simulink model "snap_adc5g_spec"  (R2019a)
settings: Solver=VariableStepDiscrete  StartTime=0.0  StopTime=10.0  RelTol=1e-3
undefined symbols (not defined in the file): pfb_coeff_gen_calc
libraries: xbsIndex_r4 x13965, casper_library_misc x80, casper_library_delays x43, xps_library x5, xbsReplacements_r4 x2, casper_library_communications x1
(part 152 of 152)

== system snap_adc5g_spec/fft_wideband_real/fft_biplex_real_4x/biplex_core/fft_stage_11/butterfly_direct/twiddle/bus_mult/mult2/b_replicate/bussify ==
  in1 : Inport
  in2 : Inport  Port=2
  concatenate : xbsIndex_r4/Concat  num_inputs=2  dbl_ovrd=off  block_type=concat
  reinterpret1 : xbsIndex_r4/Reinterpret  force_arith_type=on  arith_type=Unsigned  force_bin_pt=on  bin_pt=0  block_type=reinterpret
      settings: infoedit="Changes signal type without altering the binary representation.   You can changed the signal between signed and unsigned, and relocate the binary point.<br><br>Hardware notes: In hardware this block costs nothing.<br><br>Example:  Suppose the input is 6 bits wide, signed, with 2 fractional bits, and the output is forced to unsigned with 0 fractional bits.  Then an input of -2.0 (1110.00 in binary 2's complement) becomes an output of 56 (111000 in binary)."
  reinterpret2 : xbsIndex_r4/Reinterpret  force_arith_type=on  arith_type=Unsigned  force_bin_pt=on  bin_pt=0  block_type=reinterpret
      settings: infoedit="Changes signal type without altering the binary representation.   You can changed the signal between signed and unsigned, and relocate the binary point.<br><br>Hardware notes: In hardware this block costs nothing.<br><br>Example:  Suppose the input is 6 bits wide, signed, with 2 fractional bits, and the output is forced to unsigned with 0 fractional bits.  Then an input of -2.0 (1110.00 in binary 2's complement) becomes an output of 56 (111000 in binary)."
  bus_out : Outport
  wires:
  concatenate/1 -> bus_out/1
  in1/1 -> reinterpret1/1
  reinterpret1/1 -> concatenate/1
  in2/1 -> reinterpret2/1
  reinterpret2/1 -> concatenate/2

== system snap_adc5g_spec/fft_wideband_real/fft_biplex_real_4x/biplex_core/fft_stage_3/butterfly_direct/twiddle/bus_mult/mult1/a_replicate/bussify ==
  in1 : Inport
  in2 : Inport  Port=2
  concatenate : xbsIndex_r4/Concat  num_inputs=2  dbl_ovrd=off  block_type=concat
  reinterpret1 : xbsIndex_r4/Reinterpret  force_arith_type=on  arith_type=Unsigned  force_bin_pt=on  bin_pt=0  block_type=reinterpret
      settings: infoedit="Changes signal type without altering the binary representation.   You can changed the signal between signed and unsigned, and relocate the binary point.<br><br>Hardware notes: In hardware this block costs nothing.<br><br>Example:  Suppose the input is 6 bits wide, signed, with 2 fractional bits, and the output is forced to unsigned with 0 fractional bits.  Then an input of -2.0 (1110.00 in binary 2's complement) becomes an output of 56 (111000 in binary)."
  reinterpret2 : xbsIndex_r4/Reinterpret  force_arith_type=on  arith_type=Unsigned  force_bin_pt=on  bin_pt=0  block_type=reinterpret
      settings: infoedit="Changes signal type without altering the binary representation.   You can changed the signal between signed and unsigned, and relocate the binary point.<br><br>Hardware notes: In hardware this block costs nothing.<br><br>Example:  Suppose the input is 6 bits wide, signed, with 2 fractional bits, and the output is forced to unsigned with 0 fractional bits.  Then an input of -2.0 (1110.00 in binary 2's complement) becomes an output of 56 (111000 in binary)."
  bus_out : Outport
  wires:
  concatenate/1 -> bus_out/1
  in1/1 -> reinterpret1/1
  reinterpret1/1 -> concatenate/1
  in2/1 -> reinterpret2/1
  reinterpret2/1 -> concatenate/2

== system snap_adc5g_spec/fft_wideband_real/fft_biplex_real_4x/biplex_core/fft_stage_3/butterfly_direct/twiddle/bus_mult/mult1/b_replicate/bussify ==
  in1 : Inport
  in2 : Inport  Port=2
  concatenate : xbsIndex_r4/Concat  num_inputs=2  dbl_ovrd=off  block_type=concat
  reinterpret1 : xbsIndex_r4/Reinterpret  force_arith_type=on  arith_type=Unsigned  force_bin_pt=on  bin_pt=0  block_type=reinterpret
      settings: infoedit="Changes signal type without altering the binary representation.   You can changed the signal between signed and unsigned, and relocate the binary point.<br><br>Hardware notes: In hardware this block costs nothing.<br><br>Example:  Suppose the input is 6 bits wide, signed, with 2 fractional bits, and the output is forced to unsigned with 0 fractional bits.  Then an input of -2.0 (1110.00 in binary 2's complement) becomes an output of 56 (111000 in binary)."
  reinterpret2 : xbsIndex_r4/Reinterpret  force_arith_type=on  arith_type=Unsigned  force_bin_pt=on  bin_pt=0  block_type=reinterpret
      settings: infoedit="Changes signal type without altering the binary representation.   You can changed the signal between signed and unsigned, and relocate the binary point.<br><br>Hardware notes: In hardware this block costs nothing.<br><br>Example:  Suppose the input is 6 bits wide, signed, with 2 fractional bits, and the output is forced to unsigned with 0 fractional bits.  Then an input of -2.0 (1110.00 in binary 2's complement) becomes an output of 56 (111000 in binary)."
  bus_out : Outport
  wires:
  concatenate/1 -> bus_out/1
  in1/1 -> reinterpret1/1
  reinterpret1/1 -> concatenate/1
  in2/1 -> reinterpret2/1
  reinterpret2/1 -> concatenate/2

== system snap_adc5g_spec/fft_wideband_real/fft_biplex_real_4x/biplex_core/fft_stage_3/butterfly_direct/twiddle/bus_mult/mult2/a_replicate/bussify ==
  in1 : Inport
  in2 : Inport  Port=2
  concatenate : xbsIndex_r4/Concat  num_inputs=2  dbl_ovrd=off  block_type=concat
  reinterpret1 : xbsIndex_r4/Reinterpret  force_arith_type=on  arith_type=Unsigned  force_bin_pt=on  bin_pt=0  block_type=reinterpret
      settings: infoedit="Changes signal type without altering the binary representation.   You can changed the signal between signed and unsigned, and relocate the binary point.<br><br>Hardware notes: In hardware this block costs nothing.<br><br>Example:  Suppose the input is 6 bits wide, signed, with 2 fractional bits, and the output is forced to unsigned with 0 fractional bits.  Then an input of -2.0 (1110.00 in binary 2's complement) becomes an output of 56 (111000 in binary)."
  reinterpret2 : xbsIndex_r4/Reinterpret  force_arith_type=on  arith_type=Unsigned  force_bin_pt=on  bin_pt=0  block_type=reinterpret
      settings: infoedit="Changes signal type without altering the binary representation.   You can changed the signal between signed and unsigned, and relocate the binary point.<br><br>Hardware notes: In hardware this block costs nothing.<br><br>Example:  Suppose the input is 6 bits wide, signed, with 2 fractional bits, and the output is forced to unsigned with 0 fractional bits.  Then an input of -2.0 (1110.00 in binary 2's complement) becomes an output of 56 (111000 in binary)."
  bus_out : Outport
  wires:
  concatenate/1 -> bus_out/1
  in1/1 -> reinterpret1/1
  reinterpret1/1 -> concatenate/1
  in2/1 -> reinterpret2/1
  reinterpret2/1 -> concatenate/2

== system snap_adc5g_spec/fft_wideband_real/fft_biplex_real_4x/biplex_core/fft_stage_3/butterfly_direct/twiddle/bus_mult/mult2/b_replicate/bussify ==
  in1 : Inport
  in2 : Inport  Port=2
  concatenate : xbsIndex_r4/Concat  num_inputs=2  dbl_ovrd=off  block_type=concat
  reinterpret1 : xbsIndex_r4/Reinterpret  force_arith_type=on  arith_type=Unsigned  force_bin_pt=on  bin_pt=0  block_type=reinterpret
      settings: infoedit="Changes signal type without altering the binary representation.   You can changed the signal between signed and unsigned, and relocate the binary point.<br><br>Hardware notes: In hardware this block costs nothing.<br><br>Example:  Suppose the input is 6 bits wide, signed, with 2 fractional bits, and the output is forced to unsigned with 0 fractional bits.  Then an input of -2.0 (1110.00 in binary 2's complement) becomes an output of 56 (111000 in binary)."
  reinterpret2 : xbsIndex_r4/Reinterpret  force_arith_type=on  arith_type=Unsigned  force_bin_pt=on  bin_pt=0  block_type=reinterpret
      settings: infoedit="Changes signal type without altering the binary representation.   You can changed the signal between signed and unsigned, and relocate the binary point.<br><br>Hardware notes: In hardware this block costs nothing.<br><br>Example:  Suppose the input is 6 bits wide, signed, with 2 fractional bits, and the output is forced to unsigned with 0 fractional bits.  Then an input of -2.0 (1110.00 in binary 2's complement) becomes an output of 56 (111000 in binary)."
  bus_out : Outport
  wires:
  concatenate/1 -> bus_out/1
  in1/1 -> reinterpret1/1
  reinterpret1/1 -> concatenate/1
  in2/1 -> reinterpret2/1
  reinterpret2/1 -> concatenate/2

== system snap_adc5g_spec/fft_wideband_real/fft_biplex_real_4x/biplex_core/fft_stage_4/butterfly_direct/twiddle/bus_mult/mult1/a_replicate/bussify ==
  in1 : Inport
  in2 : Inport  Port=2
  concatenate : xbsIndex_r4/Concat  num_inputs=2  dbl_ovrd=off  block_type=concat
  reinterpret1 : xbsIndex_r4/Reinterpret  force_arith_type=on  arith_type=Unsigned  force_bin_pt=on  bin_pt=0  block_type=reinterpret
      settings: infoedit="Changes signal type without altering the binary representation.   You can changed the signal between signed and unsigned, and relocate the binary point.<br><br>Hardware notes: In hardware this block costs nothing.<br><br>Example:  Suppose the input is 6 bits wide, signed, with 2 fractional bits, and the output is forced to unsigned with 0 fractional bits.  Then an input of -2.0 (1110.00 in binary 2's complement) becomes an output of 56 (111000 in binary)."
  reinterpret2 : xbsIndex_r4/Reinterpret  force_arith_type=on  arith_type=Unsigned  force_bin_pt=on  bin_pt=0  block_type=reinterpret
      settings: infoedit="Changes signal type without altering the binary representation.   You can changed the signal between signed and unsigned, and relocate the binary point.<br><br>Hardware notes: In hardware this block costs nothing.<br><br>Example:  Suppose the input is 6 bits wide, signed, with 2 fractional bits, and the output is forced to unsigned with 0 fractional bits.  Then an input of -2.0 (1110.00 in binary 2's complement) becomes an output of 56 (111000 in binary)."
  bus_out : Outport
  wires:
  concatenate/1 -> bus_out/1
  in1/1 -> reinterpret1/1
  reinterpret1/1 -> concatenate/1
  in2/1 -> reinterpret2/1
  reinterpret2/1 -> concatenate/2

== system snap_adc5g_spec/fft_wideband_real/fft_biplex_real_4x/biplex_core/fft_stage_4/butterfly_direct/twiddle/bus_mult/mult1/b_replicate/bussify ==
  in1 : Inport
  in2 : Inport  Port=2
  concatenate : xbsIndex_r4/Concat  num_inputs=2  dbl_ovrd=off  block_type=concat
  reinterpret1 : xbsIndex_r4/Reinterpret  force_arith_type=on  arith_type=Unsigned  force_bin_pt=on  bin_pt=0  block_type=reinterpret
      settings: infoedit="Changes signal type without altering the binary representation.   You can changed the signal between signed and unsigned, and relocate the binary point.<br><br>Hardware notes: In hardware this block costs nothing.<br><br>Example:  Suppose the input is 6 bits wide, signed, with 2 fractional bits, and the output is forced to unsigned with 0 fractional bits.  Then an input of -2.0 (1110.00 in binary 2's complement) becomes an output of 56 (111000 in binary)."
  reinterpret2 : xbsIndex_r4/Reinterpret  force_arith_type=on  arith_type=Unsigned  force_bin_pt=on  bin_pt=0  block_type=reinterpret
      settings: infoedit="Changes signal type without altering the binary representation.   You can changed the signal between signed and unsigned, and relocate the binary point.<br><br>Hardware notes: In hardware this block costs nothing.<br><br>Example:  Suppose the input is 6 bits wide, signed, with 2 fractional bits, and the output is forced to unsigned with 0 fractional bits.  Then an input of -2.0 (1110.00 in binary 2's complement) becomes an output of 56 (111000 in binary)."
  bus_out : Outport
  wires:
  concatenate/1 -> bus_out/1
  in1/1 -> reinterpret1/1
  reinterpret1/1 -> concatenate/1
  in2/1 -> reinterpret2/1
  reinterpret2/1 -> concatenate/2

== system snap_adc5g_spec/fft_wideband_real/fft_biplex_real_4x/biplex_core/fft_stage_4/butterfly_direct/twiddle/bus_mult/mult2/a_replicate/bussify ==
  in1 : Inport
  in2 : Inport  Port=2
  concatenate : xbsIndex_r4/Concat  num_inputs=2  dbl_ovrd=off  block_type=concat
  reinterpret1 : xbsIndex_r4/Reinterpret  force_arith_type=on  arith_type=Unsigned  force_bin_pt=on  bin_pt=0  block_type=reinterpret
      settings: infoedit="Changes signal type without altering the binary representation.   You can changed the signal between signed and unsigned, and relocate the binary point.<br><br>Hardware notes: In hardware this block costs nothing.<br><br>Example:  Suppose the input is 6 bits wide, signed, with 2 fractional bits, and the output is forced to unsigned with 0 fractional bits.  Then an input of -2.0 (1110.00 in binary 2's complement) becomes an output of 56 (111000 in binary)."
  reinterpret2 : xbsIndex_r4/Reinterpret  force_arith_type=on  arith_type=Unsigned  force_bin_pt=on  bin_pt=0  block_type=reinterpret
      settings: infoedit="Changes signal type without altering the binary representation.   You can changed the signal between signed and unsigned, and relocate the binary point.<br><br>Hardware notes: In hardware this block costs nothing.<br><br>Example:  Suppose the input is 6 bits wide, signed, with 2 fractional bits, and the output is forced to unsigned with 0 fractional bits.  Then an input of -2.0 (1110.00 in binary 2's complement) becomes an output of 56 (111000 in binary)."
  bus_out : Outport
  wires:
  concatenate/1 -> bus_out/1
  in1/1 -> reinterpret1/1
  reinterpret1/1 -> concatenate/1
  in2/1 -> reinterpret2/1
  reinterpret2/1 -> concatenate/2

== system snap_adc5g_spec/fft_wideband_real/fft_biplex_real_4x/biplex_core/fft_stage_4/butterfly_direct/twiddle/bus_mult/mult2/b_replicate/bussify ==
  in1 : Inport
  in2 : Inport  Port=2
  concatenate : xbsIndex_r4/Concat  num_inputs=2  dbl_ovrd=off  block_type=concat
  reinterpret1 : xbsIndex_r4/Reinterpret  force_arith_type=on  arith_type=Unsigned  force_bin_pt=on  bin_pt=0  block_type=reinterpret
      settings: infoedit="Changes signal type without altering the binary representation.   You can changed the signal between signed and unsigned, and relocate the binary point.<br><br>Hardware notes: In hardware this block costs nothing.<br><br>Example:  Suppose the input is 6 bits wide, signed, with 2 fractional bits, and the output is forced to unsigned with 0 fractional bits.  Then an input of -2.0 (1110.00 in binary 2's complement) becomes an output of 56 (111000 in binary)."
  reinterpret2 : xbsIndex_r4/Reinterpret  force_arith_type=on  arith_type=Unsigned  force_bin_pt=on  bin_pt=0  block_type=reinterpret
      settings: infoedit="Changes signal type without altering the binary representation.   You can changed the signal between signed and unsigned, and relocate the binary point.<br><br>Hardware notes: In hardware this block costs nothing.<br><br>Example:  Suppose the input is 6 bits wide, signed, with 2 fractional bits, and the output is forced to unsigned with 0 fractional bits.  Then an input of -2.0 (1110.00 in binary 2's complement) becomes an output of 56 (111000 in binary)."
  bus_out : Outport
  wires:
  concatenate/1 -> bus_out/1
  in1/1 -> reinterpret1/1
  reinterpret1/1 -> concatenate/1
  in2/1 -> reinterpret2/1
  reinterpret2/1 -> concatenate/2

== system snap_adc5g_spec/fft_wideband_real/fft_biplex_real_4x/biplex_core/fft_stage_5/butterfly_direct/twiddle/bus_mult/mult1/a_replicate/bussify ==
  in1 : Inport
  in2 : Inport  Port=2
  concatenate : xbsIndex_r4/Concat  num_inputs=2  dbl_ovrd=off  block_type=concat
  reinterpret1 : xbsIndex_r4/Reinterpret  force_arith_type=on  arith_type=Unsigned  force_bin_pt=on  bin_pt=0  block_type=reinterpret
      settings: infoedit="Changes signal type without altering the binary representation.   You can changed the signal between signed and unsigned, and relocate the binary point.<br><br>Hardware notes: In hardware this block costs nothing.<br><br>Example:  Suppose the input is 6 bits wide, signed, with 2 fractional bits, and the output is forced to unsigned with 0 fractional bits.  Then an input of -2.0 (1110.00 in binary 2's complement) becomes an output of 56 (111000 in binary)."
  reinterpret2 : xbsIndex_r4/Reinterpret  force_arith_type=on  arith_type=Unsigned  force_bin_pt=on  bin_pt=0  block_type=reinterpret
      settings: infoedit="Changes signal type without altering the binary representation.   You can changed the signal between signed and unsigned, and relocate the binary point.<br><br>Hardware notes: In hardware this block costs nothing.<br><br>Example:  Suppose the input is 6 bits wide, signed, with 2 fractional bits, and the output is forced to unsigned with 0 fractional bits.  Then an input of -2.0 (1110.00 in binary 2's complement) becomes an output of 56 (111000 in binary)."
  bus_out : Outport
  wires:
  concatenate/1 -> bus_out/1
  in1/1 -> reinterpret1/1
  reinterpret1/1 -> concatenate/1
  in2/1 -> reinterpret2/1
  reinterpret2/1 -> concatenate/2

== system snap_adc5g_spec/fft_wideband_real/fft_biplex_real_4x/biplex_core/fft_stage_5/butterfly_direct/twiddle/bus_mult/mult1/b_replicate/bussify ==
  in1 : Inport
  in2 : Inport  Port=2
  concatenate : xbsIndex_r4/Concat  num_inputs=2  dbl_ovrd=off  block_type=concat
  reinterpret1 : xbsIndex_r4/Reinterpret  force_arith_type=on  arith_type=Unsigned  force_bin_pt=on  bin_pt=0  block_type=reinterpret
      settings: infoedit="Changes signal type without altering the binary representation.   You can changed the signal between signed and unsigned, and relocate the binary point.<br><br>Hardware notes: In hardware this block costs nothing.<br><br>Example:  Suppose the input is 6 bits wide, signed, with 2 fractional bits, and the output is forced to unsigned with 0 fractional bits.  Then an input of -2.0 (1110.00 in binary 2's complement) becomes an output of 56 (111000 in binary)."
  reinterpret2 : xbsIndex_r4/Reinterpret  force_arith_type=on  arith_type=Unsigned  force_bin_pt=on  bin_pt=0  block_type=reinterpret
      settings: infoedit="Changes signal type without altering the binary representation.   You can changed the signal between signed and unsigned, and relocate the binary point.<br><br>Hardware notes: In hardware this block costs nothing.<br><br>Example:  Suppose the input is 6 bits wide, signed, with 2 fractional bits, and the output is forced to unsigned with 0 fractional bits.  Then an input of -2.0 (1110.00 in binary 2's complement) becomes an output of 56 (111000 in binary)."
  bus_out : Outport
  wires:
  concatenate/1 -> bus_out/1
  in1/1 -> reinterpret1/1
  reinterpret1/1 -> concatenate/1
  in2/1 -> reinterpret2/1
  reinterpret2/1 -> concatenate/2

== system snap_adc5g_spec/fft_wideband_real/fft_biplex_real_4x/biplex_core/fft_stage_5/butterfly_direct/twiddle/bus_mult/mult2/a_replicate/bussify ==
  in1 : Inport
  in2 : Inport  Port=2
  concatenate : xbsIndex_r4/Concat  num_inputs=2  dbl_ovrd=off  block_type=concat
  reinterpret1 : xbsIndex_r4/Reinterpret  force_arith_type=on  arith_type=Unsigned  force_bin_pt=on  bin_pt=0  block_type=reinterpret
      settings: infoedit="Changes signal type without altering the binary representation.   You can changed the signal between signed and unsigned, and relocate the binary point.<br><br>Hardware notes: In hardware this block costs nothing.<br><br>Example:  Suppose the input is 6 bits wide, signed, with 2 fractional bits, and the output is forced to unsigned with 0 fractional bits.  Then an input of -2.0 (1110.00 in binary 2's complement) becomes an output of 56 (111000 in binary)."
  reinterpret2 : xbsIndex_r4/Reinterpret  force_arith_type=on  arith_type=Unsigned  force_bin_pt=on  bin_pt=0  block_type=reinterpret
      settings: infoedit="Changes signal type without altering the binary representation.   You can changed the signal between signed and unsigned, and relocate the binary point.<br><br>Hardware notes: In hardware this block costs nothing.<br><br>Example:  Suppose the input is 6 bits wide, signed, with 2 fractional bits, and the output is forced to unsigned with 0 fractional bits.  Then an input of -2.0 (1110.00 in binary 2's complement) becomes an output of 56 (111000 in binary)."
  bus_out : Outport
  wires:
  concatenate/1 -> bus_out/1
  in1/1 -> reinterpret1/1
  reinterpret1/1 -> concatenate/1
  in2/1 -> reinterpret2/1
  reinterpret2/1 -> concatenate/2

== system snap_adc5g_spec/fft_wideband_real/fft_biplex_real_4x/biplex_core/fft_stage_5/butterfly_direct/twiddle/bus_mult/mult2/b_replicate/bussify ==
  in1 : Inport
  in2 : Inport  Port=2
  concatenate : xbsIndex_r4/Concat  num_inputs=2  dbl_ovrd=off  block_type=concat
  reinterpret1 : xbsIndex_r4/Reinterpret  force_arith_type=on  arith_type=Unsigned  force_bin_pt=on  bin_pt=0  block_type=reinterpret
      settings: infoedit="Changes signal type without altering the binary representation.   You can changed the signal between signed and unsigned, and relocate the binary point.<br><br>Hardware notes: In hardware this block costs nothing.<br><br>Example:  Suppose the input is 6 bits wide, signed, with 2 fractional bits, and the output is forced to unsigned with 0 fractional bits.  Then an input of -2.0 (1110.00 in binary 2's complement) becomes an output of 56 (111000 in binary)."
  reinterpret2 : xbsIndex_r4/Reinterpret  force_arith_type=on  arith_type=Unsigned  force_bin_pt=on  bin_pt=0  block_type=reinterpret
      settings: infoedit="Changes signal type without altering the binary representation.   You can changed the signal between signed and unsigned, and relocate the binary point.<br><br>Hardware notes: In hardware this block costs nothing.<br><br>Example:  Suppose the input is 6 bits wide, signed, with 2 fractional bits, and the output is forced to unsigned with 0 fractional bits.  Then an input of -2.0 (1110.00 in binary 2's complement) becomes an output of 56 (111000 in binary)."
  bus_out : Outport
  wires:
  concatenate/1 -> bus_out/1
  in1/1 -> reinterpret1/1
  reinterpret1/1 -> concatenate/1
  in2/1 -> reinterpret2/1
  reinterpret2/1 -> concatenate/2

== system snap_adc5g_spec/fft_wideband_real/fft_biplex_real_4x/biplex_core/fft_stage_6/butterfly_direct/twiddle/bus_mult/mult1/a_replicate/bussify ==
  in1 : Inport
  in2 : Inport  Port=2
  concatenate : xbsIndex_r4/Concat  num_inputs=2  dbl_ovrd=off  block_type=concat
  reinterpret1 : xbsIndex_r4/Reinterpret  force_arith_type=on  arith_type=Unsigned  force_bin_pt=on  bin_pt=0  block_type=reinterpret
      settings: infoedit="Changes signal type without altering the binary representation.   You can changed the signal between signed and unsigned, and relocate the binary point.<br><br>Hardware notes: In hardware this block costs nothing.<br><br>Example:  Suppose the input is 6 bits wide, signed, with 2 fractional bits, and the output is forced to unsigned with 0 fractional bits.  Then an input of -2.0 (1110.00 in binary 2's complement) becomes an output of 56 (111000 in binary)."
  reinterpret2 : xbsIndex_r4/Reinterpret  force_arith_type=on  arith_type=Unsigned  force_bin_pt=on  bin_pt=0  block_type=reinterpret
      settings: infoedit="Changes signal type without altering the binary representation.   You can changed the signal between signed and unsigned, and relocate the binary point.<br><br>Hardware notes: In hardware this block costs nothing.<br><br>Example:  Suppose the input is 6 bits wide, signed, with 2 fractional bits, and the output is forced to unsigned with 0 fractional bits.  Then an input of -2.0 (1110.00 in binary 2's complement) becomes an output of 56 (111000 in binary)."
  bus_out : Outport
  wires:
  concatenate/1 -> bus_out/1
  in1/1 -> reinterpret1/1
  reinterpret1/1 -> concatenate/1
  in2/1 -> reinterpret2/1
  reinterpret2/1 -> concatenate/2

== system snap_adc5g_spec/fft_wideband_real/fft_biplex_real_4x/biplex_core/fft_stage_6/butterfly_direct/twiddle/bus_mult/mult1/b_replicate/bussify ==
  in1 : Inport
  in2 : Inport  Port=2
  concatenate : xbsIndex_r4/Concat  num_inputs=2  dbl_ovrd=off  block_type=concat
  reinterpret1 : xbsIndex_r4/Reinterpret  force_arith_type=on  arith_type=Unsigned  force_bin_pt=on  bin_pt=0  block_type=reinterpret
      settings: infoedit="Changes signal type without altering the binary representation.   You can changed the signal between signed and unsigned, and relocate the binary point.<br><br>Hardware notes: In hardware this block costs nothing.<br><br>Example:  Suppose the input is 6 bits wide, signed, with 2 fractional bits, and the output is forced to unsigned with 0 fractional bits.  Then an input of -2.0 (1110.00 in binary 2's complement) becomes an output of 56 (111000 in binary)."
  reinterpret2 : xbsIndex_r4/Reinterpret  force_arith_type=on  arith_type=Unsigned  force_bin_pt=on  bin_pt=0  block_type=reinterpret
      settings: infoedit="Changes signal type without altering the binary representation.   You can changed the signal between signed and unsigned, and relocate the binary point.<br><br>Hardware notes: In hardware this block costs nothing.<br><br>Example:  Suppose the input is 6 bits wide, signed, with 2 fractional bits, and the output is forced to unsigned with 0 fractional bits.  Then an input of -2.0 (1110.00 in binary 2's complement) becomes an output of 56 (111000 in binary)."
  bus_out : Outport
  wires:
  concatenate/1 -> bus_out/1
  in1/1 -> reinterpret1/1
  reinterpret1/1 -> concatenate/1
  in2/1 -> reinterpret2/1
  reinterpret2/1 -> concatenate/2

== system snap_adc5g_spec/fft_wideband_real/fft_biplex_real_4x/biplex_core/fft_stage_6/butterfly_direct/twiddle/bus_mult/mult2/a_replicate/bussify ==
  in1 : Inport
  in2 : Inport  Port=2
  concatenate : xbsIndex_r4/Concat  num_inputs=2  dbl_ovrd=off  block_type=concat
  reinterpret1 : xbsIndex_r4/Reinterpret  force_arith_type=on  arith_type=Unsigned  force_bin_pt=on  bin_pt=0  block_type=reinterpret
      settings: infoedit="Changes signal type without altering the binary representation.   You can changed the signal between signed and unsigned, and relocate the binary point.<br><br>Hardware notes: In hardware this block costs nothing.<br><br>Example:  Suppose the input is 6 bits wide, signed, with 2 fractional bits, and the output is forced to unsigned with 0 fractional bits.  Then an input of -2.0 (1110.00 in binary 2's complement) becomes an output of 56 (111000 in binary)."
  reinterpret2 : xbsIndex_r4/Reinterpret  force_arith_type=on  arith_type=Unsigned  force_bin_pt=on  bin_pt=0  block_type=reinterpret
      settings: infoedit="Changes signal type without altering the binary representation.   You can changed the signal between signed and unsigned, and relocate the binary point.<br><br>Hardware notes: In hardware this block costs nothing.<br><br>Example:  Suppose the input is 6 bits wide, signed, with 2 fractional bits, and the output is forced to unsigned with 0 fractional bits.  Then an input of -2.0 (1110.00 in binary 2's complement) becomes an output of 56 (111000 in binary)."
  bus_out : Outport
  wires:
  concatenate/1 -> bus_out/1
  in1/1 -> reinterpret1/1
  reinterpret1/1 -> concatenate/1
  in2/1 -> reinterpret2/1
  reinterpret2/1 -> concatenate/2

== system snap_adc5g_spec/fft_wideband_real/fft_biplex_real_4x/biplex_core/fft_stage_6/butterfly_direct/twiddle/bus_mult/mult2/b_replicate/bussify ==
  in1 : Inport
  in2 : Inport  Port=2
  concatenate : xbsIndex_r4/Concat  num_inputs=2  dbl_ovrd=off  block_type=concat
  reinterpret1 : xbsIndex_r4/Reinterpret  force_arith_type=on  arith_type=Unsigned  force_bin_pt=on  bin_pt=0  block_type=reinterpret
      settings: infoedit="Changes signal type without altering the binary representation.   You can changed the signal between signed and unsigned, and relocate the binary point.<br><br>Hardware notes: In hardware this block costs nothing.<br><br>Example:  Suppose the input is 6 bits wide, signed, with 2 fractional bits, and the output is forced to unsigned with 0 fractional bits.  Then an input of -2.0 (1110.00 in binary 2's complement) becomes an output of 56 (111000 in binary)."
  reinterpret2 : xbsIndex_r4/Reinterpret  force_arith_type=on  arith_type=Unsigned  force_bin_pt=on  bin_pt=0  block_type=reinterpret
      settings: infoedit="Changes signal type without altering the binary representation.   You can changed the signal between signed and unsigned, and relocate the binary point.<br><br>Hardware notes: In hardware this block costs nothing.<br><br>Example:  Suppose the input is 6 bits wide, signed, with 2 fractional bits, and the output is forced to unsigned with 0 fractional bits.  Then an input of -2.0 (1110.00 in binary 2's complement) becomes an output of 56 (111000 in binary)."
  bus_out : Outport
  wires:
  concatenate/1 -> bus_out/1
  in1/1 -> reinterpret1/1
  reinterpret1/1 -> concatenate/1
  in2/1 -> reinterpret2/1
  reinterpret2/1 -> concatenate/2

== system snap_adc5g_spec/fft_wideband_real/fft_biplex_real_4x/biplex_core/fft_stage_7/butterfly_direct/twiddle/bus_mult/mult1/a_replicate/bussify ==
  in1 : Inport
  in2 : Inport  Port=2
  concatenate : xbsIndex_r4/Concat  num_inputs=2  dbl_ovrd=off  block_type=concat
  reinterpret1 : xbsIndex_r4/Reinterpret  force_arith_type=on  arith_type=Unsigned  force_bin_pt=on  bin_pt=0  block_type=reinterpret
      settings: infoedit="Changes signal type without altering the binary representation.   You can changed the signal between signed and unsigned, and relocate the binary point.<br><br>Hardware notes: In hardware this block costs nothing.<br><br>Example:  Suppose the input is 6 bits wide, signed, with 2 fractional bits, and the output is forced to unsigned with 0 fractional bits.  Then an input of -2.0 (1110.00 in binary 2's complement) becomes an output of 56 (111000 in binary)."
  reinterpret2 : xbsIndex_r4/Reinterpret  force_arith_type=on  arith_type=Unsigned  force_bin_pt=on  bin_pt=0  block_type=reinterpret
      settings: infoedit="Changes signal type without altering the binary representation.   You can changed the signal between signed and unsigned, and relocate the binary point.<br><br>Hardware notes: In hardware this block costs nothing.<br><br>Example:  Suppose the input is 6 bits wide, signed, with 2 fractional bits, and the output is forced to unsigned with 0 fractional bits.  Then an input of -2.0 (1110.00 in binary 2's complement) becomes an output of 56 (111000 in binary)."
  bus_out : Outport
  wires:
  concatenate/1 -> bus_out/1
  in1/1 -> reinterpret1/1
  reinterpret1/1 -> concatenate/1
  in2/1 -> reinterpret2/1
  reinterpret2/1 -> concatenate/2

== system snap_adc5g_spec/fft_wideband_real/fft_biplex_real_4x/biplex_core/fft_stage_7/butterfly_direct/twiddle/bus_mult/mult1/b_replicate/bussify ==
  in1 : Inport
  in2 : Inport  Port=2
  concatenate : xbsIndex_r4/Concat  num_inputs=2  dbl_ovrd=off  block_type=concat
  reinterpret1 : xbsIndex_r4/Reinterpret  force_arith_type=on  arith_type=Unsigned  force_bin_pt=on  bin_pt=0  block_type=reinterpret
      settings: infoedit="Changes signal type without altering the binary representation.   You can changed the signal between signed and unsigned, and relocate the binary point.<br><br>Hardware notes: In hardware this block costs nothing.<br><br>Example:  Suppose the input is 6 bits wide, signed, with 2 fractional bits, and the output is forced to unsigned with 0 fractional bits.  Then an input of -2.0 (1110.00 in binary 2's complement) becomes an output of 56 (111000 in binary)."
  reinterpret2 : xbsIndex_r4/Reinterpret  force_arith_type=on  arith_type=Unsigned  force_bin_pt=on  bin_pt=0  block_type=reinterpret
      settings: infoedit="Changes signal type without altering the binary representation.   You can changed the signal between signed and unsigned, and relocate the binary point.<br><br>Hardware notes: In hardware this block costs nothing.<br><br>Example:  Suppose the input is 6 bits wide, signed, with 2 fractional bits, and the output is forced to unsigned with 0 fractional bits.  Then an input of -2.0 (1110.00 in binary 2's complement) becomes an output of 56 (111000 in binary)."
  bus_out : Outport
  wires:
  concatenate/1 -> bus_out/1
  in1/1 -> reinterpret1/1
  reinterpret1/1 -> concatenate/1
  in2/1 -> reinterpret2/1
  reinterpret2/1 -> concatenate/2

== system snap_adc5g_spec/fft_wideband_real/fft_biplex_real_4x/biplex_core/fft_stage_7/butterfly_direct/twiddle/bus_mult/mult2/a_replicate/bussify ==
  in1 : Inport
  in2 : Inport  Port=2
  concatenate : xbsIndex_r4/Concat  num_inputs=2  dbl_ovrd=off  block_type=concat
  reinterpret1 : xbsIndex_r4/Reinterpret  force_arith_type=on  arith_type=Unsigned  force_bin_pt=on  bin_pt=0  block_type=reinterpret
      settings: infoedit="Changes signal type without altering the binary representation.   You can changed the signal between signed and unsigned, and relocate the binary point.<br><br>Hardware notes: In hardware this block costs nothing.<br><br>Example:  Suppose the input is 6 bits wide, signed, with 2 fractional bits, and the output is forced to unsigned with 0 fractional bits.  Then an input of -2.0 (1110.00 in binary 2's complement) becomes an output of 56 (111000 in binary)."
  reinterpret2 : xbsIndex_r4/Reinterpret  force_arith_type=on  arith_type=Unsigned  force_bin_pt=on  bin_pt=0  block_type=reinterpret
      settings: infoedit="Changes signal type without altering the binary representation.   You can changed the signal between signed and unsigned, and relocate the binary point.<br><br>Hardware notes: In hardware this block costs nothing.<br><br>Example:  Suppose the input is 6 bits wide, signed, with 2 fractional bits, and the output is forced to unsigned with 0 fractional bits.  Then an input of -2.0 (1110.00 in binary 2's complement) becomes an output of 56 (111000 in binary)."
  bus_out : Outport
  wires:
  concatenate/1 -> bus_out/1
  in1/1 -> reinterpret1/1
  reinterpret1/1 -> concatenate/1
  in2/1 -> reinterpret2/1
  reinterpret2/1 -> concatenate/2

== system snap_adc5g_spec/fft_wideband_real/fft_biplex_real_4x/biplex_core/fft_stage_7/butterfly_direct/twiddle/bus_mult/mult2/b_replicate/bussify ==
  in1 : Inport
  in2 : Inport  Port=2
  concatenate : xbsIndex_r4/Concat  num_inputs=2  dbl_ovrd=off  block_type=concat
  reinterpret1 : xbsIndex_r4/Reinterpret  force_arith_type=on  arith_type=Unsigned  force_bin_pt=on  bin_pt=0  block_type=reinterpret
      settings: infoedit="Changes signal type without altering the binary representation.   You can changed the signal between signed and unsigned, and relocate the binary point.<br><br>Hardware notes: In hardware this block costs nothing.<br><br>Example:  Suppose the input is 6 bits wide, signed, with 2 fractional bits, and the output is forced to unsigned with 0 fractional bits.  Then an input of -2.0 (1110.00 in binary 2's complement) becomes an output of 56 (111000 in binary)."
  reinterpret2 : xbsIndex_r4/Reinterpret  force_arith_type=on  arith_type=Unsigned  force_bin_pt=on  bin_pt=0  block_type=reinterpret
      settings: infoedit="Changes signal type without altering the binary representation.   You can changed the signal between signed and unsigned, and relocate the binary point.<br><br>Hardware notes: In hardware this block costs nothing.<br><br>Example:  Suppose the input is 6 bits wide, signed, with 2 fractional bits, and the output is forced to unsigned with 0 fractional bits.  Then an input of -2.0 (1110.00 in binary 2's complement) becomes an output of 56 (111000 in binary)."
  bus_out : Outport
  wires:
  concatenate/1 -> bus_out/1
  in1/1 -> reinterpret1/1
  reinterpret1/1 -> concatenate/1
  in2/1 -> reinterpret2/1
  reinterpret2/1 -> concatenate/2

== system snap_adc5g_spec/fft_wideband_real/fft_biplex_real_4x/biplex_core/fft_stage_8/butterfly_direct/twiddle/bus_mult/mult1/a_replicate/bussify ==
  in1 : Inport
  in2 : Inport  Port=2
  concatenate : xbsIndex_r4/Concat  num_inputs=2  dbl_ovrd=off  block_type=concat
  reinterpret1 : xbsIndex_r4/Reinterpret  force_arith_type=on  arith_type=Unsigned  force_bin_pt=on  bin_pt=0  block_type=reinterpret
      settings: infoedit="Changes signal type without altering the binary representation.   You can changed the signal between signed and unsigned, and relocate the binary point.<br><br>Hardware notes: In hardware this block costs nothing.<br><br>Example:  Suppose the input is 6 bits wide, signed, with 2 fractional bits, and the output is forced to unsigned with 0 fractional bits.  Then an input of -2.0 (1110.00 in binary 2's complement) becomes an output of 56 (111000 in binary)."
  reinterpret2 : xbsIndex_r4/Reinterpret  force_arith_type=on  arith_type=Unsigned  force_bin_pt=on  bin_pt=0  block_type=reinterpret
      settings: infoedit="Changes signal type without altering the binary representation.   You can changed the signal between signed and unsigned, and relocate the binary point.<br><br>Hardware notes: In hardware this block costs nothing.<br><br>Example:  Suppose the input is 6 bits wide, signed, with 2 fractional bits, and the output is forced to unsigned with 0 fractional bits.  Then an input of -2.0 (1110.00 in binary 2's complement) becomes an output of 56 (111000 in binary)."
  bus_out : Outport
  wires:
  concatenate/1 -> bus_out/1
  in1/1 -> reinterpret1/1
  reinterpret1/1 -> concatenate/1
  in2/1 -> reinterpret2/1
  reinterpret2/1 -> concatenate/2

== system snap_adc5g_spec/fft_wideband_real/fft_biplex_real_4x/biplex_core/fft_stage_8/butterfly_direct/twiddle/bus_mult/mult1/b_replicate/bussify ==
  in1 : Inport
  in2 : Inport  Port=2
  concatenate : xbsIndex_r4/Concat  num_inputs=2  dbl_ovrd=off  block_type=concat
  reinterpret1 : xbsIndex_r4/Reinterpret  force_arith_type=on  arith_type=Unsigned  force_bin_pt=on  bin_pt=0  block_type=reinterpret
      settings: infoedit="Changes signal type without altering the binary representation.   You can changed the signal between signed and unsigned, and relocate the binary point.<br><br>Hardware notes: In hardware this block costs nothing.<br><br>Example:  Suppose the input is 6 bits wide, signed, with 2 fractional bits, and the output is forced to unsigned with 0 fractional bits.  Then an input of -2.0 (1110.00 in binary 2's complement) becomes an output of 56 (111000 in binary)."
  reinterpret2 : xbsIndex_r4/Reinterpret  force_arith_type=on  arith_type=Unsigned  force_bin_pt=on  bin_pt=0  block_type=reinterpret
      settings: infoedit="Changes signal type without altering the binary representation.   You can changed the signal between signed and unsigned, and relocate the binary point.<br><br>Hardware notes: In hardware this block costs nothing.<br><br>Example:  Suppose the input is 6 bits wide, signed, with 2 fractional bits, and the output is forced to unsigned with 0 fractional bits.  Then an input of -2.0 (1110.00 in binary 2's complement) becomes an output of 56 (111000 in binary)."
  bus_out : Outport
  wires:
  concatenate/1 -> bus_out/1
  in1/1 -> reinterpret1/1
  reinterpret1/1 -> concatenate/1
  in2/1 -> reinterpret2/1
  reinterpret2/1 -> concatenate/2

== system snap_adc5g_spec/fft_wideband_real/fft_biplex_real_4x/biplex_core/fft_stage_8/butterfly_direct/twiddle/bus_mult/mult2/a_replicate/bussify ==
  in1 : Inport
  in2 : Inport  Port=2
  concatenate : xbsIndex_r4/Concat  num_inputs=2  dbl_ovrd=off  block_type=concat
  reinterpret1 : xbsIndex_r4/Reinterpret  force_arith_type=on  arith_type=Unsigned  force_bin_pt=on  bin_pt=0  block_type=reinterpret
      settings: infoedit="Changes signal type without altering the binary representation.   You can changed the signal between signed and unsigned, and relocate the binary point.<br><br>Hardware notes: In hardware this block costs nothing.<br><br>Example:  Suppose the input is 6 bits wide, signed, with 2 fractional bits, and the output is forced to unsigned with 0 fractional bits.  Then an input of -2.0 (1110.00 in binary 2's complement) becomes an output of 56 (111000 in binary)."
  reinterpret2 : xbsIndex_r4/Reinterpret  force_arith_type=on  arith_type=Unsigned  force_bin_pt=on  bin_pt=0  block_type=reinterpret
      settings: infoedit="Changes signal type without altering the binary representation.   You can changed the signal between signed and unsigned, and relocate the binary point.<br><br>Hardware notes: In hardware this block costs nothing.<br><br>Example:  Suppose the input is 6 bits wide, signed, with 2 fractional bits, and the output is forced to unsigned with 0 fractional bits.  Then an input of -2.0 (1110.00 in binary 2's complement) becomes an output of 56 (111000 in binary)."
  bus_out : Outport
  wires:
  concatenate/1 -> bus_out/1
  in1/1 -> reinterpret1/1
  reinterpret1/1 -> concatenate/1
  in2/1 -> reinterpret2/1
  reinterpret2/1 -> concatenate/2

== system snap_adc5g_spec/fft_wideband_real/fft_biplex_real_4x/biplex_core/fft_stage_8/butterfly_direct/twiddle/bus_mult/mult2/b_replicate/bussify ==
  in1 : Inport
  in2 : Inport  Port=2
  concatenate : xbsIndex_r4/Concat  num_inputs=2  dbl_ovrd=off  block_type=concat
  reinterpret1 : xbsIndex_r4/Reinterpret  force_arith_type=on  arith_type=Unsigned  force_bin_pt=on  bin_pt=0  block_type=reinterpret
      settings: infoedit="Changes signal type without altering the binary representation.   You can changed the signal between signed and unsigned, and relocate the binary point.<br><br>Hardware notes: In hardware this block costs nothing.<br><br>Example:  Suppose the input is 6 bits wide, signed, with 2 fractional bits, and the output is forced to unsigned with 0 fractional bits.  Then an input of -2.0 (1110.00 in binary 2's complement) becomes an output of 56 (111000 in binary)."
  reinterpret2 : xbsIndex_r4/Reinterpret  force_arith_type=on  arith_type=Unsigned  force_bin_pt=on  bin_pt=0  block_type=reinterpret
      settings: infoedit="Changes signal type without altering the binary representation.   You can changed the signal between signed and unsigned, and relocate the binary point.<br><br>Hardware notes: In hardware this block costs nothing.<br><br>Example:  Suppose the input is 6 bits wide, signed, with 2 fractional bits, and the output is forced to unsigned with 0 fractional bits.  Then an input of -2.0 (1110.00 in binary 2's complement) becomes an output of 56 (111000 in binary)."
  bus_out : Outport
  wires:
  concatenate/1 -> bus_out/1
  in1/1 -> reinterpret1/1
  reinterpret1/1 -> concatenate/1
  in2/1 -> reinterpret2/1
  reinterpret2/1 -> concatenate/2

== system snap_adc5g_spec/fft_wideband_real/fft_biplex_real_4x/biplex_core/fft_stage_9/butterfly_direct/twiddle/bus_mult/mult1/a_replicate/bussify ==
  in1 : Inport
  in2 : Inport  Port=2
  concatenate : xbsIndex_r4/Concat  num_inputs=2  dbl_ovrd=off  block_type=concat
  reinterpret1 : xbsIndex_r4/Reinterpret  force_arith_type=on  arith_type=Unsigned  force_bin_pt=on  bin_pt=0  block_type=reinterpret
      settings: infoedit="Changes signal type without altering the binary representation.   You can changed the signal between signed and unsigned, and relocate the binary point.<br><br>Hardware notes: In hardware this block costs nothing.<br><br>Example:  Suppose the input is 6 bits wide, signed, with 2 fractional bits, and the output is forced to unsigned with 0 fractional bits.  Then an input of -2.0 (1110.00 in binary 2's complement) becomes an output of 56 (111000 in binary)."
  reinterpret2 : xbsIndex_r4/Reinterpret  force_arith_type=on  arith_type=Unsigned  force_bin_pt=on  bin_pt=0  block_type=reinterpret
      settings: infoedit="Changes signal type without altering the binary representation.   You can changed the signal between signed and unsigned, and relocate the binary point.<br><br>Hardware notes: In hardware this block costs nothing.<br><br>Example:  Suppose the input is 6 bits wide, signed, with 2 fractional bits, and the output is forced to unsigned with 0 fractional bits.  Then an input of -2.0 (1110.00 in binary 2's complement) becomes an output of 56 (111000 in binary)."
  bus_out : Outport
  wires:
  concatenate/1 -> bus_out/1
  in1/1 -> reinterpret1/1
  reinterpret1/1 -> concatenate/1
  in2/1 -> reinterpret2/1
  reinterpret2/1 -> concatenate/2

== system snap_adc5g_spec/fft_wideband_real/fft_biplex_real_4x/biplex_core/fft_stage_9/butterfly_direct/twiddle/bus_mult/mult1/b_replicate/bussify ==
  in1 : Inport
  in2 : Inport  Port=2
  concatenate : xbsIndex_r4/Concat  num_inputs=2  dbl_ovrd=off  block_type=concat
  reinterpret1 : xbsIndex_r4/Reinterpret  force_arith_type=on  arith_type=Unsigned  force_bin_pt=on  bin_pt=0  block_type=reinterpret
      settings: infoedit="Changes signal type without altering the binary representation.   You can changed the signal between signed and unsigned, and relocate the binary point.<br><br>Hardware notes: In hardware this block costs nothing.<br><br>Example:  Suppose the input is 6 bits wide, signed, with 2 fractional bits, and the output is forced to unsigned with 0 fractional bits.  Then an input of -2.0 (1110.00 in binary 2's complement) becomes an output of 56 (111000 in binary)."
  reinterpret2 : xbsIndex_r4/Reinterpret  force_arith_type=on  arith_type=Unsigned  force_bin_pt=on  bin_pt=0  block_type=reinterpret
      settings: infoedit="Changes signal type without altering the binary representation.   You can changed the signal between signed and unsigned, and relocate the binary point.<br><br>Hardware notes: In hardware this block costs nothing.<br><br>Example:  Suppose the input is 6 bits wide, signed, with 2 fractional bits, and the output is forced to unsigned with 0 fractional bits.  Then an input of -2.0 (1110.00 in binary 2's complement) becomes an output of 56 (111000 in binary)."
  bus_out : Outport
  wires:
  concatenate/1 -> bus_out/1
  in1/1 -> reinterpret1/1
  reinterpret1/1 -> concatenate/1
  in2/1 -> reinterpret2/1
  reinterpret2/1 -> concatenate/2

== system snap_adc5g_spec/fft_wideband_real/fft_biplex_real_4x/biplex_core/fft_stage_9/butterfly_direct/twiddle/bus_mult/mult2/a_replicate/bussify ==
  in1 : Inport
  in2 : Inport  Port=2
  concatenate : xbsIndex_r4/Concat  num_inputs=2  dbl_ovrd=off  block_type=concat
  reinterpret1 : xbsIndex_r4/Reinterpret  force_arith_type=on  arith_type=Unsigned  force_bin_pt=on  bin_pt=0  block_type=reinterpret
      settings: infoedit="Changes signal type without altering the binary representation.   You can changed the signal between signed and unsigned, and relocate the binary point.<br><br>Hardware notes: In hardware this block costs nothing.<br><br>Example:  Suppose the input is 6 bits wide, signed, with 2 fractional bits, and the output is forced to unsigned with 0 fractional bits.  Then an input of -2.0 (1110.00 in binary 2's complement) becomes an output of 56 (111000 in binary)."
  reinterpret2 : xbsIndex_r4/Reinterpret  force_arith_type=on  arith_type=Unsigned  force_bin_pt=on  bin_pt=0  block_type=reinterpret
      settings: infoedit="Changes signal type without altering the binary representation.   You can changed the signal between signed and unsigned, and relocate the binary point.<br><br>Hardware notes: In hardware this block costs nothing.<br><br>Example:  Suppose the input is 6 bits wide, signed, with 2 fractional bits, and the output is forced to unsigned with 0 fractional bits.  Then an input of -2.0 (1110.00 in binary 2's complement) becomes an output of 56 (111000 in binary)."
  bus_out : Outport
  wires:
  concatenate/1 -> bus_out/1
  in1/1 -> reinterpret1/1
  reinterpret1/1 -> concatenate/1
  in2/1 -> reinterpret2/1
  reinterpret2/1 -> concatenate/2

== system snap_adc5g_spec/fft_wideband_real/fft_biplex_real_4x/biplex_core/fft_stage_9/butterfly_direct/twiddle/bus_mult/mult2/b_replicate/bussify ==
  in1 : Inport
  in2 : Inport  Port=2
  concatenate : xbsIndex_r4/Concat  num_inputs=2  dbl_ovrd=off  block_type=concat
  reinterpret1 : xbsIndex_r4/Reinterpret  force_arith_type=on  arith_type=Unsigned  force_bin_pt=on  bin_pt=0  block_type=reinterpret
      settings: infoedit="Changes signal type without altering the binary representation.   You can changed the signal between signed and unsigned, and relocate the binary point.<br><br>Hardware notes: In hardware this block costs nothing.<br><br>Example:  Suppose the input is 6 bits wide, signed, with 2 fractional bits, and the output is forced to unsigned with 0 fractional bits.  Then an input of -2.0 (1110.00 in binary 2's complement) becomes an output of 56 (111000 in binary)."
  reinterpret2 : xbsIndex_r4/Reinterpret  force_arith_type=on  arith_type=Unsigned  force_bin_pt=on  bin_pt=0  block_type=reinterpret
      settings: infoedit="Changes signal type without altering the binary representation.   You can changed the signal between signed and unsigned, and relocate the binary point.<br><br>Hardware notes: In hardware this block costs nothing.<br><br>Example:  Suppose the input is 6 bits wide, signed, with 2 fractional bits, and the output is forced to unsigned with 0 fractional bits.  Then an input of -2.0 (1110.00 in binary 2's complement) becomes an output of 56 (111000 in binary)."
  bus_out : Outport
  wires:
  concatenate/1 -> bus_out/1
  in1/1 -> reinterpret1/1
  reinterpret1/1 -> concatenate/1
  in2/1 -> reinterpret2/1
  reinterpret2/1 -> concatenate/2
